simulink model "CartPendulumControl"  (R2025b)
settings: Solver=ode45  StartTime=0.0  StopTime=10  MaxStep=0.01  RelTol=1e-8  AbsTol=1e-10
values from neighbouring files (symbols this model uses):
  A = [0 1 0 0; g/Lp 0 0 0; 0 0 0 1; 0 0 0 0]    [build_pendulum_model.m]    (also in pendulum_project.m)
  alpha0 = 0.5    [build_pendulum_model.m]    (also in pendulum_project.m)
  amax = 0.5    [build_pendulum_model.m]    (also in pendulum_project.m)
  B = [0; -1/Lp; 0; 1]    [build_pendulum_model.m]    (also in pendulum_project.m)
  C = [1 0 0 0; 0 0 1 0]    [build_pendulum_model.m]    (also in pendulum_project.m)
  g = 9.81    [build_pendulum_model.m]    (also in pendulum_project.m)
  K = Kf(1:4)    [build_pendulum_model.m]    (also in pendulum_project.m)
  Ki = -Kf(5)    [build_pendulum_model.m]    (also in pendulum_project.m)
  Lo = place(A', C', po)'    [build_pendulum_model.m]    (also in pendulum_project.m)
  Lp = 0.5    [build_pendulum_model.m]    (also in pendulum_project.m)
  r = 1    [build_pendulum_model.m]    (also in pendulum_project.m)
settings Model: Creator=Barknar  LastModifiedBy=Barknar
settings DataIOCC: SaveFormat=Array

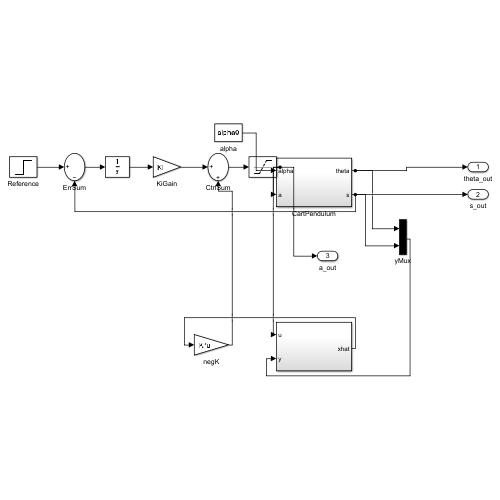
[thumbnail: Simulink's stored preview of the top-level diagram]
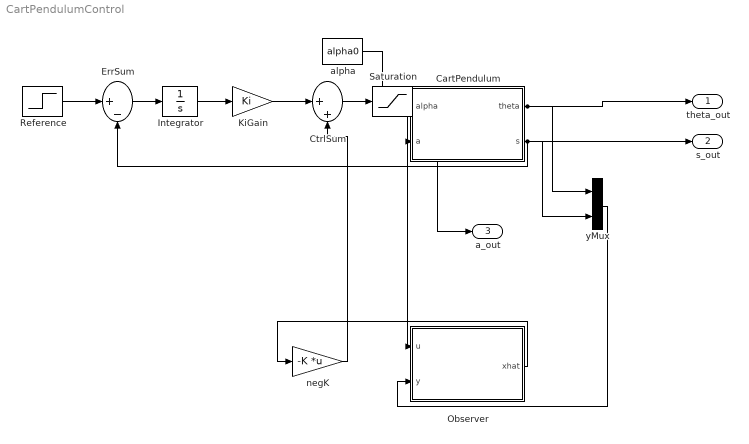
== system CartPendulumControl ==
  CartPendulum : Subsystem
  CtrlSum : Sum  Inputs=|++
  ErrSum : Sum  Inputs=|+-
  Integrator : Integrator
  KiGain : Gain  Gain=Ki
  Observer : Subsystem
  Reference : Step  Time=0  After=r  SampleTime=0
  Saturation : Saturate  UpperLimit=amax  LowerLimit=-amax
  alpha : Constant  Value=alpha0
  negK : Gain  Gain=-K  Multiplication=Matrix(K*u)
  yMux : Mux  Inputs=[1 1]
  theta_out : Outport
  s_out : Outport  Port=2
  a_out : Outport  Port=3
  wires:
  Reference/1 -> ErrSum/1
  ErrSum/1 -> Integrator/1
  Integrator/1 -> KiGain/1
  KiGain/1 -> CtrlSum/1
  negK/1 -> CtrlSum/2
  CtrlSum/1 -> Saturation/1
  alpha/1 -> CartPendulum/1(alpha)
  Saturation/1 -> CartPendulum/2(a), Observer/1(u), a_out/1
  CartPendulum/1(theta) -> yMux/1, theta_out/1
  CartPendulum/2(s) -> yMux/2, ErrSum/2, s_out/1
  yMux/1 -> Observer/2(y)
  Observer/1(xhat) -> negK/1

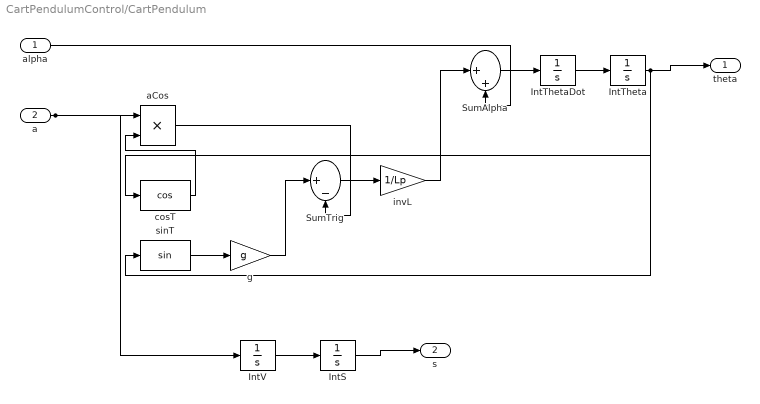
== system CartPendulumControl/CartPendulum ==
  alpha : Inport
  a : Inport  Port=2
  IntS : Integrator
  IntTheta : Integrator
  IntThetaDot : Integrator
  IntV : Integrator
  SumAlpha : Sum  Inputs=|++
  SumTrig : Sum  Inputs=|+-
  aCos : Product
  cosT : Trigonometry  Operator=cos
  g : Gain  Gain=g
  invL : Gain  Gain=1/Lp
  sinT : Trigonometry
  theta : Outport
  s : Outport  Port=2
  wires:
  a/1 -> aCos/1, IntV/1
  cosT/1 -> aCos/2
  sinT/1 -> g/1
  g/1 -> SumTrig/1
  aCos/1 -> SumTrig/2
  SumTrig/1 -> invL/1
  invL/1 -> SumAlpha/1
  alpha/1 -> SumAlpha/2
  SumAlpha/1 -> IntThetaDot/1
  IntThetaDot/1 -> IntTheta/1
  IntTheta/1 -> sinT/1, cosT/1, theta/1
  IntV/1 -> IntS/1
  IntS/1 -> s/1

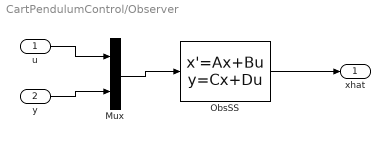
== system CartPendulumControl/Observer ==
  u : Inport
  y : Inport  Port=2
  Mux : Mux  Inputs=[1 2]
  ObsSS : StateSpace  A=A-Lo*C  B=[B Lo]  C=eye(4)  D=zeros(4,3)  InitialCondition=0
  xhat : Outport
  wires:
  u/1 -> Mux/1
  y/1 -> Mux/2
  Mux/1 -> ObsSS/1
  ObsSS/1 -> xhat/1
